simulink model "QDrone_YOLO_Recenter_Integration_Test"  (R2021b)
settings: Solver=ode2  StartTime=0.0  StopTime=60  FixedStep=0.001  RelTol=1e-3  EnableMultiTasking=on
undefined symbols (not defined in the file): Host, qc_get_step_size
libraries: quarc_library x32, simulink x5, dspnetwork x1
(part 1 of 2)
settings Model: SimulationMode=external  ExtModeTrigDuration=10000  Creator=Admin  LastModifiedBy=user
settings SolverCC: AlgebraicLoopSolver=TrustRegion  PositivePriorityOrder=on
settings DataIOCC: ReturnWorkspaceOutputs=off
settings DebuggingCC: SFUnexpectedBacktrackingDiag=warning  SFNoUnconditionalDefaultTransitionDiag=warning  SFExecutionAtInitializationDiag=none  SFMachineParentedDataDiag=warning  ArithmeticOperatorsInVariantConditions=warning
settings SFSimCC: SimUseLocalCustomCode=off  CustomCodeUndefinedFunction=UseInterfaceOnly
settings RTWCC: Description=QUARC Win64 Target Using Toolchain  SystemTargetFile=quarc_win64.tlc  TemplateMakefile=quarc_default_tmf  RTWUseLocalCustomCode=off  Toolchain=QUARC win64 | nmake (64-bit Windows)  BuildConfiguration=Faster Runs
settings CodeAppCC: StateflowObjectComments=on
settings STFCustomTargetCC: ConcurrentExecutionCompliant=on  UseToolchainInfoCompliant=on  SystemTargetFile=quarc_win64.tlc
settings GRTTargetCC: TargetLangStandard=C89/C90 (ANSI)  ParMdlRefBuildCompliant=off  CompOptLevelCompliant=off  CombineOutputUpdateFcns=off  MatFileLogging=off  CPPClassGenCompliant=off  GRTInterface=on  ExtMode=on  ExtModeMexFile=quarc_comm  ExtModeMexArgs='-w -d %d -uri %u -URI_Leader tcpip://localhost:18001 -URI_Follower tcpip://localhost:18002'
settings ConfigComp: CovMetricSettings=dw  CovSaveCumulativeToWorkspaceVar=on  CovSaveSingleToWorkspaceVar=on  CovExternalEMLEnable=off

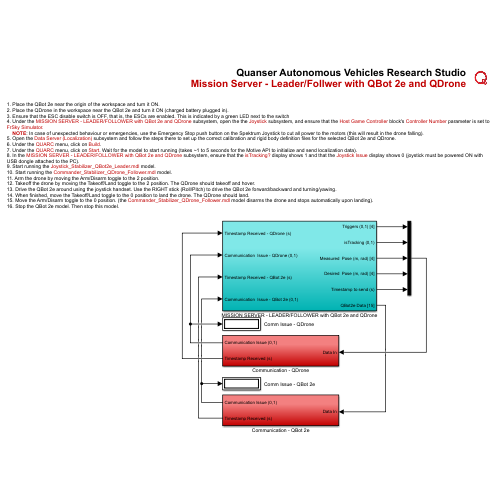
[thumbnail: Simulink's stored preview of the top-level diagram]
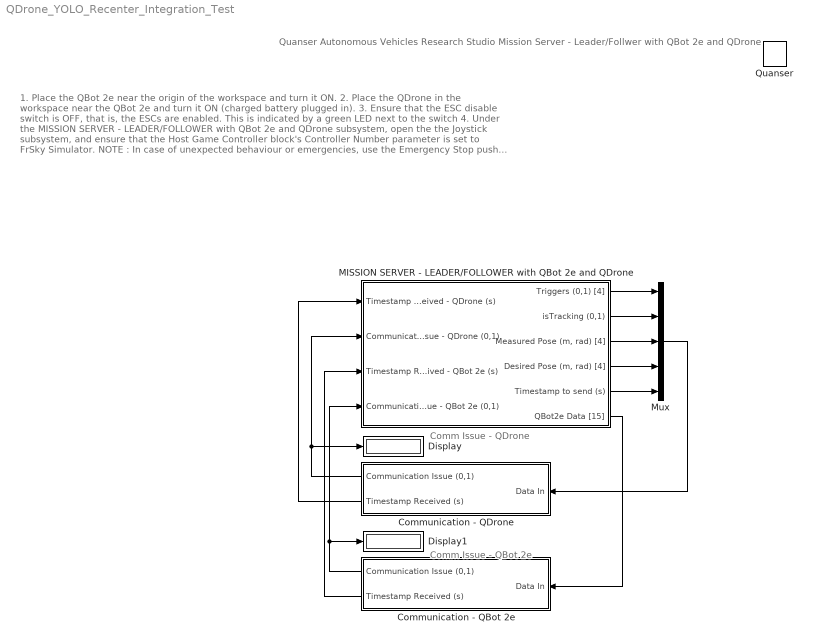
== system QDrone_YOLO_Recenter_Integration_Test ==
  note: 1. Place the QBot 2e near the origin of the workspace and turn it ON.
      | 2. Place the QDrone in the workspace near the QBot 2e and turn it ON (charged battery plugged in).
      | 3. Ensure that the ESC disable switch is OFF, that is, the ESCs are enabled. This is indicated by a green LED next to the switch
      | 4. Under the MISSION SERVER - LEADER/FOLLOWER with QBot 2e and QDrone subsystem, open the the Joystick subsystem, and ensure that the Host Game Controller block's Controller Number parameter is set to FrSky Simulator.
      | NOTE : In case of unexpected behaviour or emergencies, use the Emergency Stop push button on the Spektrum Joystick to cut all power to the motors (this will result in the drone falling).
      | 5. Open the Data Server (Localization) subsystem and follow the steps there to set up the correct calibration and rigid body definition files for the selected QBot 2e and QDrone.
      | 6. Under the QUARC menu, click on Build .
      | 7. Under the QUARC menu, click on Start . Wait for the model to start running (takes ~1 to 5 seconds for the Motive API to initialize and send localization data).
      | 8. In the MISSION SERVER - LEADER/FOLLOWER with QBot 2e and QDrone subsystem, ensure that the isTracking? display shows 1 and that the Joystick Issue display shows 0 (joystick must be powered ON with USB dongle attached to the PC).
      | 9. Start running the Joystick_Stabilizer_QBot2e_Leader.mdl model.
      | 10. Start running the Commander_Stabilizer_QDrone_Follower.mdl model.
      | 11. Arm the drone by moving the Arm/Disarm toggle to the 2 position.
      | 12. Takeoff the drone by moving the Takeoff/Land toggle to the 2 position. The QDrone should takeoff and hover.
      | 13. Drive the QBot 2e around using the joystick handset. Use the RIGHT stick (Roll/Pitch) to drive the QBot 2e forward/backward and turning/yawing.
      | 14. When finished, move the Takeoff/Land toggle to the 0 position to land the drone. The QDrone should land.
      | 15. Move the Arm/Disarm toggle to the 0 position. (the Commander_Stabilizer_QDrone_Follower.mdl model disarms the drone and stops automatically upon landing).
      | 16. Stop the QBot 2e model. Then stop this model.
  note: Quanser Autonomous Vehicles Research Studio
      | Mission Server - Leader/Follwer with QBot 2e and QDrone
  note: Comm Issue - QDrone
  note: Comm Issue - QBot 2e
  Communication - QBot 2e : Subsystem
  Communication - QDrone : Subsystem
  Display : Display
  Display1 : Display
  MISSION SERVER - LEADER/FOLLOWER with QBot 2e and QDrone : Subsystem
  Mux : Mux  Inputs=5
  Quanser : quarc_library/Logos/Quanser
  wires:
  Communication - QDrone/2(Timestamp Received (s)) -> MISSION SERVER - LEADER/FOLLOWER with QBot 2e and QDrone/1(Timestamp Received - QDrone (s))
  MISSION SERVER - LEADER/FOLLOWER with QBot 2e and QDrone/5(Timestamp to send (s)) -> Mux/5
  Mux/1 -> Communication - QDrone/1(Data In)
  Communication - QDrone/1(Communication Issue (0,1)) -> Display/1, MISSION SERVER - LEADER/FOLLOWER with QBot 2e and QDrone/2(Communication Issue - QDrone (0,1))
  MISSION SERVER - LEADER/FOLLOWER with QBot 2e and QDrone/3("Measured Pose (m, rad) [4]") -> Mux/3
  MISSION SERVER - LEADER/FOLLOWER with QBot 2e and QDrone/4("Desired Pose (m, rad) [4]") -> Mux/4
  Communication - QBot 2e/1(Communication Issue (0,1)) -> MISSION SERVER - LEADER/FOLLOWER with QBot 2e and QDrone/4(Communication Issue - QBot 2e (0,1)), Display1/1
  Communication - QBot 2e/2(Timestamp Received (s)) -> MISSION SERVER - LEADER/FOLLOWER with QBot 2e and QDrone/3(Timestamp Received - QBot 2e (s))
  MISSION SERVER - LEADER/FOLLOWER with QBot 2e and QDrone/6(QBot2e Data [15]) -> Communication - QBot 2e/1(Data In)
  MISSION SERVER - LEADER/FOLLOWER with QBot 2e and QDrone/1(Triggers (0,1) [4]) -> Mux/1
  MISSION SERVER - LEADER/FOLLOWER with QBot 2e and QDrone/2(isTracking (0,1)) -> Mux/2

== system QDrone_YOLO_Recenter_Integration_Test/Communication - QBot 2e ==
  note: Argument (URI_Leader) is set at the MEX-file arguments found at Model Configuration Properties > Code Generation > Interface
      |
      | Format:
      | tcpip://localhost:18001
  Data In : Inport
  Constant : Constant
  Detect Communication loss : Subsystem
  Model Argument : quarc_library/Sources/Signals/Model Argument  argument_name=URI_Leader  has_value=on  data_type_mode=Specify via dialog  data_type=char  max_length=80  default_value=0  variable_size=off
      settings: AttributesFormatString=(-%<argument_name>)  SourceProductName=QUARC Targets
  Stream Server : quarc_library/Communications/Basic/Stream Server  uri_source=External input port  uri=tcpip://localhost:18877  send_buffer_size=1460  receive_buffer_size=1460  byte_order=little endian (Intel - LSB first)  optimization=Minimum latency  send_options=Send most recent data  receive_options=Receive most recent data  default_value=[0]  sample_time=qc_get_step_size  active=off  implementation=Use blocking I/O in a separate thread  send_fifo_size=1000  receive_fifo_size=1000  send_priority=0  receive_priority=0  send_dimensions=off  receive_dimensions=off  max_dimensions=-1  data_type=Inherited via back propagation  type_expr=BusObject
  "String Display " : quarc_library/Strings/String Display  alignment=center  display_mode=Single line  sample_time=-1  use_new=off
      settings: SourceProductName=QUARC Targets
  Terminator1 : Terminator
  Terminator2 : Terminator
  Communication Issue (0,1) : Outport  VectorParamsAs1DForOutWhenUnconnected=off
  Timestamp Received (s) : Outport  Port=2  VectorParamsAs1DForOutWhenUnconnected=off
  wires:
  Detect Communication loss/1(Communication Issue (0,1)) -> Communication Issue (0,1)/1
  Stream Server/2 -> Detect Communication loss/2(Error)
  Stream Server/1 -> Detect Communication loss/1(State)
  Stream Server/4 -> Timestamp Received (s)/1
  Model Argument/1 -> Stream Server/3, "String Display "/1
  Stream Server/5 -> Terminator1/1
  Stream Server/3 -> Terminator2/1
  Constant/1 -> Stream Server/2
  Data In/1 -> Stream Server/1

== system QDrone_YOLO_Recenter_Integration_Test/Communication - QDrone ==
  note: Argument (URI_Follower) is set at the MEX-file arguments found at Model Configuration Properties > Code Generation > Interface
      |
      | Format:
      | tcpip://localhost:18002
  Data In : Inport
  Constant : Constant
  Detect Communication loss : Subsystem
  Model Argument : quarc_library/Sources/Signals/Model Argument  argument_name=URI_Follower  has_value=on  data_type_mode=Specify via dialog  data_type=char  max_length=80  default_value=0  variable_size=off
      settings: AttributesFormatString=(-%<argument_name>)  SourceProductName=QUARC Targets
  Stream Server : quarc_library/Communications/Basic/Stream Server  uri_source=External input port  uri=tcpip://localhost:18877  send_buffer_size=1460  receive_buffer_size=1460  byte_order=little endian (Intel - LSB first)  optimization=Minimum latency  send_options=Send most recent data  receive_options=Receive most recent data  default_value=zeros(1,1)  sample_time=qc_get_step_size  active=off  implementation=Use blocking I/O in a separate thread  send_fifo_size=1000  receive_fifo_size=1000  send_priority=0  receive_priority=0  send_dimensions=off  receive_dimensions=off  max_dimensions=-1  data_type=Inherited via back propagation  type_expr=BusObject
  "String Display " : quarc_library/Strings/String Display  alignment=center  display_mode=Single line  sample_time=-1  use_new=off
      settings: SourceProductName=QUARC Targets
  Terminator1 : Terminator
  Terminator2 : Terminator
  Communication Issue (0,1) : Outport  VectorParamsAs1DForOutWhenUnconnected=off
  Timestamp Received (s) : Outport  Port=2  VectorParamsAs1DForOutWhenUnconnected=off
  wires:
  Constant/1 -> Stream Server/2
  Data In/1 -> Stream Server/1
  Stream Server/3 -> Terminator2/1
  Stream Server/5 -> Terminator1/1
  Model Argument/1 -> "String Display "/1, Stream Server/3
  Stream Server/4 -> Timestamp Received (s)/1
  Stream Server/1 -> Detect Communication loss/1(State)
  Stream Server/2 -> Detect Communication loss/2(Error)
  Detect Communication loss/1(Communication Issue (0,1)) -> Communication Issue (0,1)/1

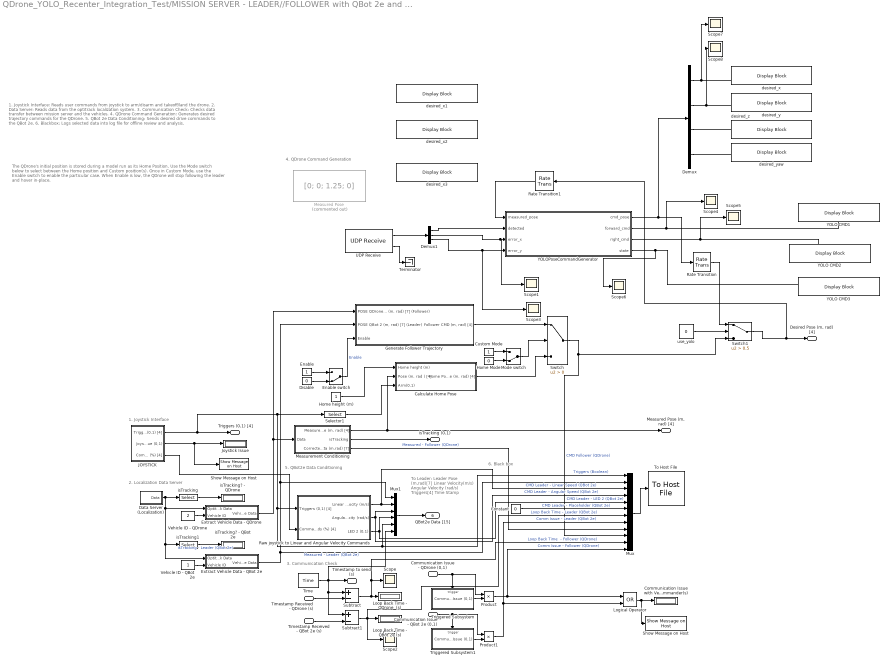
== system QDrone_YOLO_Recenter_Integration_Test/MISSION SERVER - LEADER//FOLLOWER with QBot 2e and QDrone ==
  note: To Leader:
      | Leader Pose (m,rad)[7]
      | Linear Velocity(m/s)
      | Angular Velocity (rad/s)
      | Triggers[4]
      | Time Stamp
  note: 5. QBot2e Data Conditioning
  note: The QDrone's initial position is stored during a model run as its Home Position.
      | Use the Mode switch below to select between the Home position and Custom position(s).
      | Once in Custom Mode, use the Enable switch to enable the particular case.
      | When Enable is low, the QDrone will stop following the leader and hover in-place.
  note: 3. Communication Check
  note: 6. Black box
  note: 2. Localization Data Server
  note: 1. Joystick Interface
  note: 4. QDrone Command Generation
  note: 1. Joystick Interface: Reads user commands from joystick to arm/disarm and takeoff/land the drone.
      | 2. Data Server: Reads data from the optitrack localization system.
      | 3. Communication Check: Checks data transfer between mission server and the vehicles.
      | 4. QDrone Command Generation: Generates desired trajectory commands for the QDrone.
      | 5. QBot 2e Data Conditioning: Sends desired drive commands to the QBot 2e.
      | 6. Blackbox: Logs selected data into log file for offline review and analysis.
  Timestamp Received - QDrone (s) : Inport
  Communication Issue - QDrone (0,1) : Inport  Port=2
  Timestamp Received - QBot 2e (s) : Inport  Port=3
  Communication Issue - QBot 2e (0,1) : Inport  Port=4
   desired_x{,1..3} (4 alike) : DisplayBlock  LabelPosition=Hide  Format=short  Transparency=1
  Calculate Home Pose : Subsystem
  Communication Issue with Vehicle Commander(s) : Display
  Constant : Constant  Value=0
  Custom Mode : Constant
  "Data Server (Localization) " : Subsystem
  Demux : Demux
  Demux1 : Demux  Outputs=3
  Disable : Constant  Value=0
  Enable : Constant
  Enable switch : ManualSwitch  CurrentSetting=0
  Extract Vehicle Data - QBot 2e : Subsystem
  Extract Vehicle Data - QDrone : Subsystem
  Generate Follower Trajectory : Subsystem
  Home Mode : Constant  Value=0
  Home height (m) : Constant
  JOYSTICK : Subsystem
  Joystick Issue : Display
  Logical Operator : Logic  Operator=OR  AllPortsSameDT=off  OutDataTypeStr=boolean
  Loop Back Time - QBot 2e (s) : Display
  Loop Back Time - QDrone  (s) : Display
  Measured Pose : Constant  Commented=on  Value=[0; 0; 1.25; 0]  OutDataTypeStr=double
  Measurement Conditioning : Subsystem
  Mode switch : ManualSwitch  CurrentSetting=0
  Mux : Mux  Inputs=12
  Mux1 : Mux  Inputs=6
  Product : Product
  Product1 : Product
  Rate Transition : RateTransition  OutPortSampleTime=0.001
  Rate Transition1 : RateTransition  OutPortSampleTime=0.033
  Raw joystick to Linear and Angular Velocity Commands : Subsystem
  Scope{,1..8} (9 alike) : Scope
  Selector1 : Selector  InputPortWidth=4  IndexOptions=Index vector (dialog)  Indices=[1]  OutputSizes=1
  Show Message on Host : quarc_library/Sinks/Error Handling/Show Message on Host  message_type=Fixed error message  message_icon=Warning  message=Mission Server: Communication Issue with remote vehicle(s)
      settings: AttributesFormatString="\"%<message>\""  SourceProductName=QUARC Targets
  "Show Message on Host " : quarc_library/Sinks/Error Handling/Show Message on Host  message_type=Fixed error message  message_icon=Warning  message=Mission Server: Joystick Disconnected
      settings: AttributesFormatString="\"%<message>\""  SourceProductName=QUARC Targets
  Subtract : Sum  Inputs=+-
  Subtract1 : Sum  Inputs=+-
  Switch : Switch  Criteria=u2 > Threshold
  Switch1 : Switch  Criteria=u2 > Threshold  Threshold=0.5
  Terminator : Terminator
  Time : quarc_library/Sources/Time/Time  time_source=Wall clock  sample_time=qc_get_step_size
  To Host File : quarc_library/Sinks/To Host/To Host File  file_name=saved_data/%m/Mission_Server_%{date}_%{time}.mat  variable_name=mission_server_data  decimation=1  sample_time=-1  file_format=MAT-file v.5  options=No header or footer  append=off  final_file_name=saved_data/QDrone_YOLO_Recenter_Integration_Test/Mission_Server_03-Jun-2026_14-38-11.mat  bitrate=2000000
  Triggered Subsystem : Subsystem  TreatAsAtomicUnit=on
  Triggered Subsystem1 : Subsystem  TreatAsAtomicUnit=on
  UDP Receive : dspnetwork/UDP Receive  localURL='0.0.0.0'  localPort=5010  remoteURL='0.0.0.0'  remotePort=-1  recvBufferSize=8192  dims=3  signalDatatype=double  isComplex=off  isVarSize=off  showBlockingTime=off  blockingTime=0  sampletime=0.033  blockPlatform=[]
  Vehicle ID - QBot 2e : Constant
  Vehicle ID - QDrone : Constant  Value=2
  YOLO CMD1 : DisplayBlock  LabelPosition=Hide  Format=short  Transparency=1
  YOLO CMD2 : DisplayBlock  LabelPosition=Hide  Format=short  Transparency=1
  YOLO CMD3 : DisplayBlock  LabelPosition=Hide  Format=short  Transparency=1
  YOLOPoseCommandGenerator : MATLAB Function  TreatAsAtomicUnit=on
  desired_y : DisplayBlock  LabelPosition=Hide  Format=short  Transparency=1
  "desired_yaw " : DisplayBlock  LabelPosition=Hide  Format=short  Transparency=1
  "desired_z " : DisplayBlock  LabelPosition=Hide  Format=short  Transparency=1
  isTracking : Selector  InputPortWidth=14  IndexOptions=Index vector (dialog)  Indices=[14]  OutputSizes=1
  isTracking1 : Selector  InputPortWidth=14  IndexOptions=Index vector (dialog)  Indices=[13]  OutputSizes=1
  isTracking? - QBot 2e : Display
  isTracking? - QDrone : Display
  use_yolo : Constant  Value=0
  Triggers (0,1) [4] : Outport  VectorParamsAs1DForOutWhenUnconnected=off
  isTracking (0,1) : Outport  Port=2  VectorParamsAs1DForOutWhenUnconnected=off
  "Measured Pose (m, rad) [4]" : Outport  Port=3  VectorParamsAs1DForOutWhenUnconnected=off
  "Desired Pose (m, rad) [4]" : Outport  Port=4  VectorParamsAs1DForOutWhenUnconnected=off
  Timestamp to send (s) : Outport  Port=5  VectorParamsAs1DForOutWhenUnconnected=off
  QBot2e Data [15] : Outport  Port=6  VectorParamsAs1DForOutWhenUnconnected=off
  wires:
  Communication Issue - QDrone (0,1)/1 -> Product/1, Triggered Subsystem/Trigger
  isTracking/1 -> isTracking? - QDrone/1
  JOYSTICK/2(Joystick Issue (0,1)) -> Joystick Issue/1, "Show Message on Host "/1
  Time/1 -> Mux1/6, Subtract1/1, Subtract/1, Timestamp to send (s)/1
  Timestamp Received - QDrone (s)/1 -> Subtract/2
  Subtract/1 -> Mux/11, Scope/1, Loop Back Time - QDrone  (s)/1  "Loop Back Time  - Follower (QDrone)"
  Switch/1 -> Mux/10, Switch1/3  "CMD Follower (QDrone)"
  Measurement Conditioning/2(isTracking) -> isTracking (0,1)/1
  Measurement Conditioning/1("Measured Pose (m, rad) [4]") -> "Measured Pose (m, rad) [4]"/1, Calculate Home Pose/2("Pose (m, rad ) [4]")
  "Data Server (Localization) "/1(Data) -> isTracking1/1, Extract Vehicle Data - QBot 2e/1(Optitrack Data), Extract Vehicle Data - QDrone/1(Optitrack Data), isTracking/1
  Vehicle ID - QDrone/1 -> Extract Vehicle Data - QDrone/2(Vehicle ID)
  Calculate Home Pose/1("Home Pose (m, rad) [4]") -> Switch/3
  Home height (m)/1 -> Calculate Home Pose/1(Home height (m))
  Triggered Subsystem/1(Communication Issue (0,1)) -> Product/2
  Product/1 -> Logical Operator/1, Mux/12  "Comm Issue - Follower (QDrone)"
  Mux/1 -> To Host File/1
  Custom Mode/1 -> Mode switch/1
  Mode switch/1 -> Switch/2
  Home Mode/1 -> Mode switch/2
  Enable/1 -> Enable switch/1
  Disable/1 -> Enable switch/2
  Enable switch/1 -> Generate Follower Trajectory/3(Enable)  "Enable"
  Generate Follower Trajectory/1("Follower CMD (m, rad) [4]") -> Switch/1
  Vehicle ID - QBot 2e/1 -> Extract Vehicle Data - QBot 2e/2(Vehicle ID)
  Timestamp Received - QBot 2e (s)/1 -> Subtract1/2
  Subtract1/1 -> Mux/7, Loop Back Time - QBot 2e (s)/1, Scope2/1  "Loop Back Time - Leader (QBot 2e)"
  Logical Operator/1 -> Show Message on Host/1, Communication Issue with Vehicle Commander(s)/1
  Product1/1 -> Logical Operator/2, Mux/8  "Comm Issue - Leader (QBot 2e)"
  Triggered Subsystem1/1(Communication Issue (0,1)) -> Product1/2
  Communication Issue - QBot 2e (0,1)/1 -> Product1/1, Triggered Subsystem1/Trigger
  Extract Vehicle Data - QBot 2e/1(Vehicle Data) -> Mux/2, Generate Follower Trajectory/2("POSE QBot 2 (m, rad) [7] (Leader)"), Mux1/1  "Measured - Leader (QBot 2e)"
  Extract Vehicle Data - QDrone/1(Vehicle Data) -> Measurement Conditioning/1(Data), Generate Follower Trajectory/1("POSE QDrone (m, rad) [7] (Follower)")
  isTracking1/1 -> isTracking? - QBot 2e/1  "isTracking - Leader (QBot 2e)"
  JOYSTICK/1(Triggers (0,1) [4]) -> Triggers (0,1) [4]/1, Selector1/1, Raw joystick to Linear and Angular Velocity Commands/1(Triggers (0,1) [4]), Mux/1, Mux1/5  "Triggers (Boolean)"
  Mux1/1 -> QBot2e Data [15]/1
  JOYSTICK/3(Commands (%) [4]) -> Raw joystick to Linear and Angular Velocity Commands/2(Commands (%) [4])
  Raw joystick to Linear and Angular Velocity Commands/1(Linear Velocity (m/s)) -> Mux/3, Mux1/2  "CMD Leader - Linear Speed (QBot 2e)"
  Raw joystick to Linear and Angular Velocity Commands/2(Angular Velocity (rad/s)) -> Mux1/3, Mux/4  "CMD Leader - Angular Speed (QBot 2e)"
  Raw joystick to Linear and Angular Velocity Commands/3(LED 2 (0,1)) -> Mux/5, Mux1/4  "CMD Leader - LED 2 (QBot 2e)"
  Selector1/1 -> Calculate Home Pose/3(Arm(0,1))
  Measurement Conditioning/3(Corrected Pose Data (m,rad) [7]) -> Mux/9  "Measured - Follower (QDrone)"
  Constant/1 -> Mux/6  "CMD Leader - Placeholder (QBot 2e)"
  Demux/4 -> ?
  Demux/2 -> Scope8/1
  Demux/3 -> ?
  YOLOPoseCommandGenerator/1(cmd_pose) -> Demux/1, Rate Transition/1
  use_yolo/1 -> Switch1/2
  Switch1/1 -> Rate Transition1/1, "Desired Pose (m, rad) [4]"/1
  UDP Receive/1 -> Demux1/1
  Demux1/2 -> YOLOPoseCommandGenerator/3(error_x), Scope1/1
  Demux1/3 -> YOLOPoseCommandGenerator/4(error_y), Scope3/1
  UDP Receive/2 -> Terminator/1
  Rate Transition/1 -> Switch1/1
  Rate Transition1/1 -> YOLOPoseCommandGenerator/1(measured_pose)
  YOLOPoseCommandGenerator/2(forward_cmd) -> Scope4/1
  YOLOPoseCommandGenerator/3(right_cmd) -> Scope5/1
  YOLOPoseCommandGenerator/4(state) -> Scope6/1
  Demux/1 -> Scope7/1
  Demux1/1 -> YOLOPoseCommandGenerator/2(detected)

== system QDrone_YOLO_Recenter_Integration_Test/Communication - QBot 2e/Detect Communication loss ==
  note: Check if stream is 2 (connected) and error is positive (error codes are negative). Otherwise issue a communication error.
  State : Inport
  Error : Inport  Port=2
  Data Type Conversion : DataTypeConversion
  MATLAB Function : MATLAB Function  TreatAsAtomicUnit=on
  Terminator2 : Terminator
  Threshold : quarc_library/Discontinuities/Threshold  operator=>=  param_src=Specify via dialog  threshold=0.5  duration=0.1
      settings: SourceProductName=QUARC Targets
  Time : quarc_library/Sources/Time/Time  time_source=Wall clock  sample_time=qc_get_step_size
  Communication Issue (0,1) : Outport  VectorParamsAs1DForOutWhenUnconnected=off
  wires:
  Threshold/1 -> Data Type Conversion/1
  Data Type Conversion/1 -> Communication Issue (0,1)/1
  Threshold/2 -> Terminator2/1
  Time/1 -> MATLAB Function/1(time)
  State/1 -> MATLAB Function/2(state)
  MATLAB Function/1(stream_connection_loss) -> Threshold/1
  Error/1 -> MATLAB Function/3(error)

== system QDrone_YOLO_Recenter_Integration_Test/Communication - QDrone/Detect Communication loss ==
  note: Check if stream is 2 (connected) and error is positive (error codes are negative). Otherwise issue a communication error.
  State : Inport
  Error : Inport  Port=2
  Data Type Conversion : DataTypeConversion
  MATLAB Function : MATLAB Function  TreatAsAtomicUnit=on
  Terminator2 : Terminator
  Threshold : quarc_library/Discontinuities/Threshold  operator=>=  param_src=Specify via dialog  threshold=0.5  duration=0.1
      settings: SourceProductName=QUARC Targets
  Time : quarc_library/Sources/Time/Time  time_source=Wall clock  sample_time=qc_get_step_size
  Communication Issue (0,1) : Outport  VectorParamsAs1DForOutWhenUnconnected=off
  wires:
  Error/1 -> MATLAB Function/3(error)
  MATLAB Function/1(stream_connection_loss) -> Threshold/1
  State/1 -> MATLAB Function/2(state)
  Time/1 -> MATLAB Function/1(time)
  Threshold/2 -> Terminator2/1
  Data Type Conversion/1 -> Communication Issue (0,1)/1
  Threshold/1 -> Data Type Conversion/1

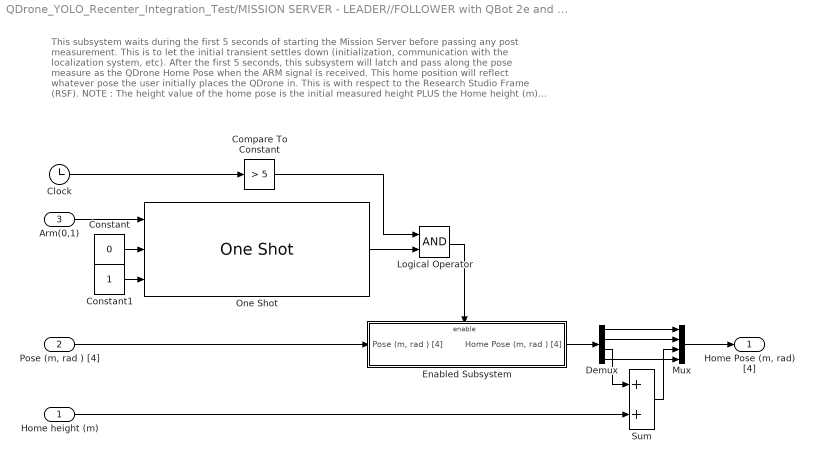
== system QDrone_YOLO_Recenter_Integration_Test/MISSION SERVER - LEADER//FOLLOWER with QBot 2e and QDrone/Calculate Home Pose ==
  note: This subsystem waits during the first 5 seconds of starting the Mission Server before passing any post measurement.
      | This is to let the initial transient settles down (initialization, communication with the localization system, etc).
      | After the first 5 seconds, this subsystem will latch and pass along the pose measure as the QDrone Home Pose when
      | the ARM signal is received.
      | This home position will reflect whatever pose the user initially places the QDrone in.
      | This is with respect to the Research Studio Frame (RSF).
      |
      | NOTE : The height value of the home pose is the initial measured height PLUS the Home height (m) input value.
  Home height (m) : Inport
  "Pose (m, rad ) [4]" : Inport  Port=2
  Arm(0,1) : Inport  Port=3
  Clock : Clock
  Compare To Constant : simulink/Logic and Bit Operations/Compare To Constant  relop=>  const=5  OutDataTypeStr=boolean
  Constant : Constant  Value=0
  Constant1 : Constant
  Demux : Demux
  Enabled Subsystem : Subsystem  TreatAsAtomicUnit=on
  Logical Operator : Logic  AllPortsSameDT=off  OutDataTypeStr=boolean
  Mux : Mux
  One Shot : quarc_library/Discontinuities/One Shot  trigger_type=Rising edge  redun_pulse=Ignore extraneous pulse  width_source=Specify via dialog  pulse_width=1/qc_get_step_size
      settings: SourceProductName=QUARC Targets
  Sum : Sum
  "Home Pose (m, rad) [4]" : Outport  VectorParamsAs1DForOutWhenUnconnected=off
  wires:
  Constant/1 -> One Shot/2
  Constant1/1 -> One Shot/3
  Arm(0,1)/1 -> One Shot/1
  One Shot/1 -> Logical Operator/2
  "Pose (m, rad ) [4]"/1 -> Enabled Subsystem/1("Pose (m, rad ) [4] ")
  Clock/1 -> Compare To Constant/1
  Compare To Constant/1 -> Logical Operator/1
  Logical Operator/1 -> Enabled Subsystem/Enable
  Enabled Subsystem/1("Home Pose (m, rad ) [4]") -> Demux/1
  Demux/1 -> Mux/1
  Demux/2 -> Mux/2
  Demux/4 -> Mux/4
  Demux/3 -> Sum/1
  Sum/1 -> Mux/3
  Home height (m)/1 -> Sum/2
  Mux/1 -> "Home Pose (m, rad) [4]"/1

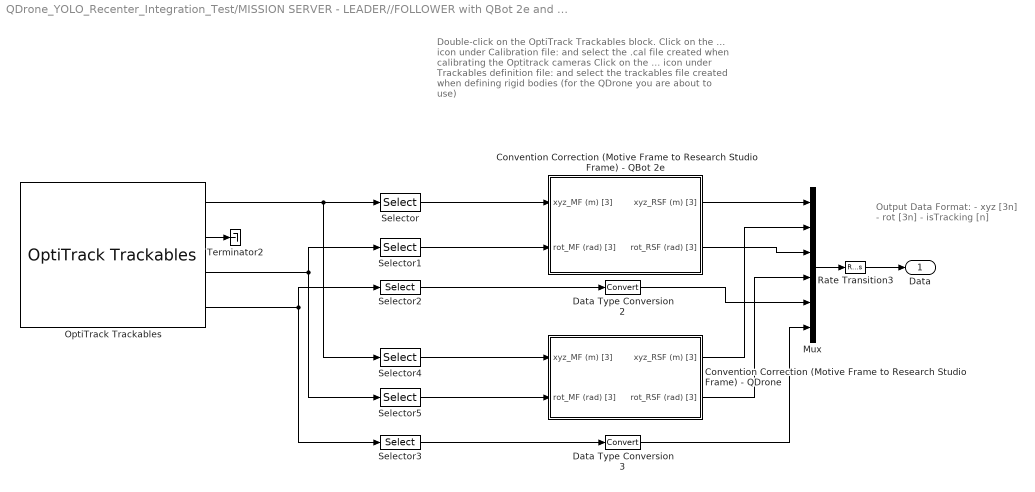
== system QDrone_YOLO_Recenter_Integration_Test/MISSION SERVER - LEADER//FOLLOWER with QBot 2e and QDrone/Data Server (Localization)  ==
  note: Output Data Format:
      | - xyz [3n]
      | - rot [3n]
      | - isTracking [n]
  note: Double-click on the OptiTrack Trackables block.
      |
      | Click on the ... icon under Calibration file: and select the .cal file
      | created when calibrating the Optitrack cameras
      |
      | Click on the ... icon under Trackables definition file: and select
      | the trackables file created when defining rigid bodies (for the
      | QDrone you are about to use)
  Convention Correction (Motive Frame to Research Studio Frame) - QBot 2e : Subsystem
  Convention Correction (Motive Frame to Research Studio Frame) - QDrone : Subsystem
  Data Type Conversion2 : DataTypeConversion
  Data Type Conversion3 : DataTypeConversion
  Mux : Mux  Inputs=6
  OptiTrack Trackables : quarc_library/Devices/Third-Party/NaturalPoint/OptiTrack/OptiTrack Trackables  calibration_file=C:\Users\user\Documents\OptiTrack\2023-05-04\Calibration Exceptional (MeanErr 0.642 mm) 2023-05-04 12.cal  rigid_body_file=C:\Users\user\Documents\OptiTrack\2023-05-04\RigidBody 02.tra  rigid_body_ids=[1,2]  sample_time=qc_get_step_size*10  active=off
      settings: SourceProductName=QUARC Targets
  Rate Transition3 : RateTransition
  Selector : Selector  InputPortWidth=6  IndexOptions=Index vector (dialog)  Indices=[1:3]  OutputSizes=1
  Selector1 : Selector  InputPortWidth=6  IndexOptions=Index vector (dialog)  Indices=[1:3]  OutputSizes=1
  Selector2 : Selector  InputPortWidth=2  IndexOptions=Index vector (dialog)  Indices=[1]  OutputSizes=1
  Selector3 : Selector  InputPortWidth=2  IndexOptions=Index vector (dialog)  Indices=[2]  OutputSizes=1
  Selector4 : Selector  InputPortWidth=6  IndexOptions=Index vector (dialog)  Indices=[4:6]  OutputSizes=1
  Selector5 : Selector  InputPortWidth=6  IndexOptions=Index vector (dialog)  Indices=[4:6]  OutputSizes=1
  Terminator2 : Terminator
  Data : Outport  VectorParamsAs1DForOutWhenUnconnected=off
  wires:
  Convention Correction (Motive Frame to Research Studio Frame) - QBot 2e/1(xyz_RSF (m) [3]) -> Mux/1
  Data Type Conversion2/1 -> Mux/5
  Convention Correction (Motive Frame to Research Studio Frame) - QBot 2e/2(rot_RSF (rad) [3]) -> Mux/3
  OptiTrack Trackables/2 -> Terminator2/1
  Data Type Conversion3/1 -> Mux/6
  Convention Correction (Motive Frame to Research Studio Frame) - QDrone/2(rot_RSF (rad) [3]) -> Mux/4
  OptiTrack Trackables/4 -> Selector2/1, Selector3/1
  Convention Correction (Motive Frame to Research Studio Frame) - QDrone/1(xyz_RSF (m) [3]) -> Mux/2
  OptiTrack Trackables/3 -> Selector5/1, Selector1/1
  Selector1/1 -> Convention Correction (Motive Frame to Research Studio Frame) - QBot 2e/2(rot_MF (rad) [3])
  Selector2/1 -> Data Type Conversion2/1
  Selector3/1 -> Data Type Conversion3/1
  OptiTrack Trackables/1 -> Selector4/1, Selector/1
  Selector/1 -> Convention Correction (Motive Frame to Research Studio Frame) - QBot 2e/1(xyz_MF (m) [3])
  Selector4/1 -> Convention Correction (Motive Frame to Research Studio Frame) - QDrone/1(xyz_MF (m) [3])
  Selector5/1 -> Convention Correction (Motive Frame to Research Studio Frame) - QDrone/2(rot_MF (rad) [3])
  Mux/1 -> Rate Transition3/1
  Rate Transition3/1 -> Data/1

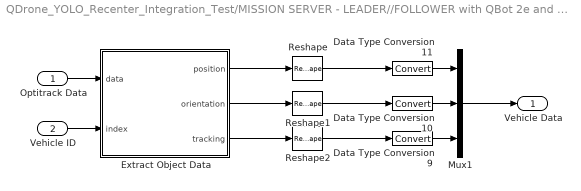
== system QDrone_YOLO_Recenter_Integration_Test/MISSION SERVER - LEADER//FOLLOWER with QBot 2e and QDrone/Extract Vehicle Data - QBot 2e ==
  Optitrack Data : Inport
  Vehicle ID : Inport  Port=2
  Data Type Conversion10 : DataTypeConversion
  Data Type Conversion11 : DataTypeConversion
  Data Type Conversion9 : DataTypeConversion
  Extract Object Data : MATLAB Function  TreatAsAtomicUnit=on
  Mux1 : Mux  Inputs=3
  Reshape : Reshape
  Reshape1 : Reshape
  Reshape2 : Reshape
  Vehicle Data : Outport  VectorParamsAs1DForOutWhenUnconnected=off
  wires:
  Reshape2/1 -> Data Type Conversion9/1
  Reshape1/1 -> Data Type Conversion10/1
  Reshape/1 -> Data Type Conversion11/1
  Data Type Conversion9/1 -> Mux1/3
  Data Type Conversion10/1 -> Mux1/2
  Data Type Conversion11/1 -> Mux1/1
  Extract Object Data/2(orientation) -> Reshape1/1
  Extract Object Data/3(tracking) -> Reshape2/1
  Extract Object Data/1(position) -> Reshape/1
  Mux1/1 -> Vehicle Data/1
  Optitrack Data/1 -> Extract Object Data/1(data)
  Vehicle ID/1 -> Extract Object Data/2(index)

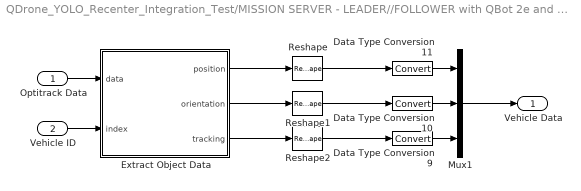
== system QDrone_YOLO_Recenter_Integration_Test/MISSION SERVER - LEADER//FOLLOWER with QBot 2e and QDrone/Extract Vehicle Data - QDrone ==
  Optitrack Data : Inport
  Vehicle ID : Inport  Port=2
  Data Type Conversion10 : DataTypeConversion
  Data Type Conversion11 : DataTypeConversion
  Data Type Conversion9 : DataTypeConversion
  Extract Object Data : MATLAB Function  TreatAsAtomicUnit=on
  Mux1 : Mux  Inputs=3
  Reshape : Reshape
  Reshape1 : Reshape
  Reshape2 : Reshape
  Vehicle Data : Outport  VectorParamsAs1DForOutWhenUnconnected=off
  wires:
  Reshape2/1 -> Data Type Conversion9/1
  Reshape1/1 -> Data Type Conversion10/1
  Reshape/1 -> Data Type Conversion11/1
  Data Type Conversion9/1 -> Mux1/3
  Data Type Conversion10/1 -> Mux1/2
  Data Type Conversion11/1 -> Mux1/1
  Extract Object Data/2(orientation) -> Reshape1/1
  Extract Object Data/3(tracking) -> Reshape2/1
  Extract Object Data/1(position) -> Reshape/1
  Mux1/1 -> Vehicle Data/1
  Optitrack Data/1 -> Extract Object Data/1(data)
  Vehicle ID/1 -> Extract Object Data/2(index)

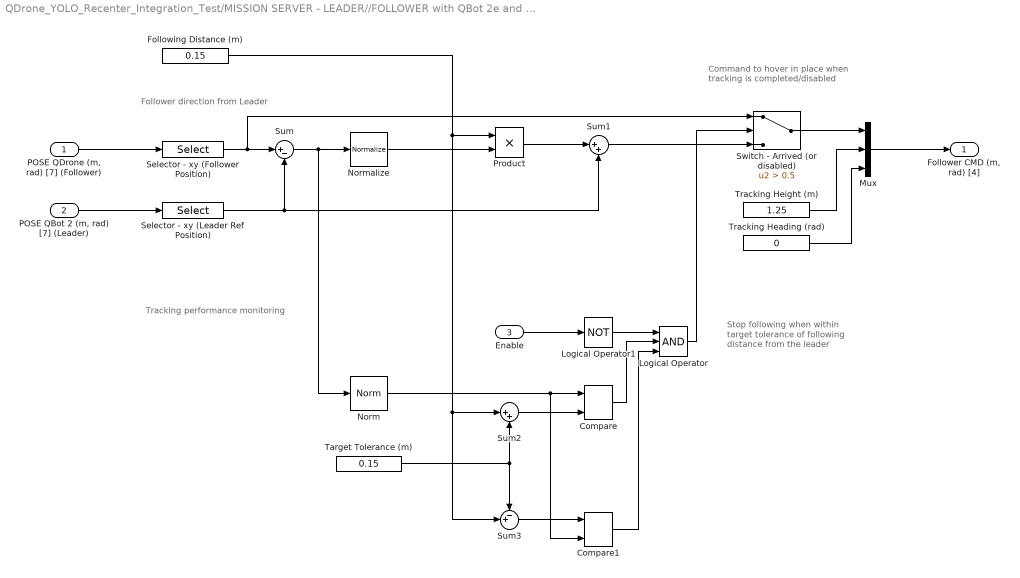
== system QDrone_YOLO_Recenter_Integration_Test/MISSION SERVER - LEADER//FOLLOWER with QBot 2e and QDrone/Generate Follower Trajectory ==
  note: Command to hover in place when
      | tracking is completed/disabled
  note: Stop following when
      | within target tolerance
      | of following distance from
      | the leader
  note: Tracking performance monitoring
  note: Follower direction from Leader
  "POSE QDrone (m, rad) [7] (Follower)" : Inport
  "POSE QBot 2 (m, rad) [7] (Leader)" : Inport  Port=2
  Enable : Inport  Port=3
  Compare : quarc_library/Logic Operations/Compare  operator=<=  output_data_type=boolean
      settings: SourceProductName=QUARC Targets
  Compare1 : quarc_library/Logic Operations/Compare  operator=>=  output_data_type=boolean
      settings: SourceProductName=QUARC Targets
  Following Distance (m) : Constant  Value=0.15
  Logical Operator : Logic  Inputs=3  AllPortsSameDT=off  OutDataTypeStr=boolean
  Logical Operator1 : Logic  Operator=NOT  Inputs=1  AllPortsSameDT=off  OutDataTypeStr=boolean
  Mux : Mux  Inputs=3
  Norm : quarc_library/Math Operations/Vectors/Norm
      settings: SourceProductName=QUARC Targets
  Normalize : quarc_library/Math Operations/Vectors/Normalize
      settings: SourceProductName=QUARC Targets
  Product : Product
  Selector - xy (Follower Position) : Selector  InputPortWidth=7  IndexOptions=Index vector (dialog)  Indices=[1 2]  OutputSizes=1
  Selector - xy (Leader Ref Position) : Selector  InputPortWidth=7  IndexOptions=Index vector (dialog)  Indices=[1 2]  OutputSizes=1
  Sum : Sum  Inputs=|+-
  Sum1 : Sum  Inputs=|++
  Sum2 : Sum  Inputs=|++
  Sum3 : Sum  Inputs=-+|
  Switch - Arrived (or disabled) : Switch  Criteria=u2 > Threshold  Threshold=0.5
  Target Tolerance (m) : Constant  Value=0.15
  Tracking Heading (rad) : Constant  Value=0
  Tracking Height (m) : Constant  Value=1.25
  "Follower CMD (m, rad) [4]" : Outport  VectorParamsAs1DForOutWhenUnconnected=off
  wires:
  "POSE QDrone (m, rad) [7] (Follower)"/1 -> Selector - xy (Follower Position)/1
  "POSE QBot 2 (m, rad) [7] (Leader)"/1 -> Selector - xy (Leader Ref Position)/1
  Selector - xy (Follower Position)/1 -> Switch - Arrived (or disabled)/1, Sum/1
  Selector - xy (Leader Ref Position)/1 -> Sum1/2, Sum/2
  Sum/1 -> Norm/1, Normalize/1
  Product/1 -> Sum1/1
  Normalize/1 -> Product/2
  Following Distance (m)/1 -> Product/1, Sum2/1, Sum3/2
  Tracking Height (m)/1 -> Mux/2
  Tracking Heading (rad)/1 -> Mux/3
  Sum1/1 -> Switch - Arrived (or disabled)/3
  Switch - Arrived (or disabled)/1 -> Mux/1
  Mux/1 -> "Follower CMD (m, rad) [4]"/1
  Sum2/1 -> Compare/2
  Sum3/1 -> Compare1/1
  Target Tolerance (m)/1 -> Sum2/2, Sum3/1
  Norm/1 -> Compare1/2, Compare/1
  Enable/1 -> Logical Operator1/1
  Logical Operator1/1 -> Logical Operator/1
  Compare/1 -> Logical Operator/2
  Compare1/1 -> Logical Operator/3
  Logical Operator/1 -> Switch - Arrived (or disabled)/2

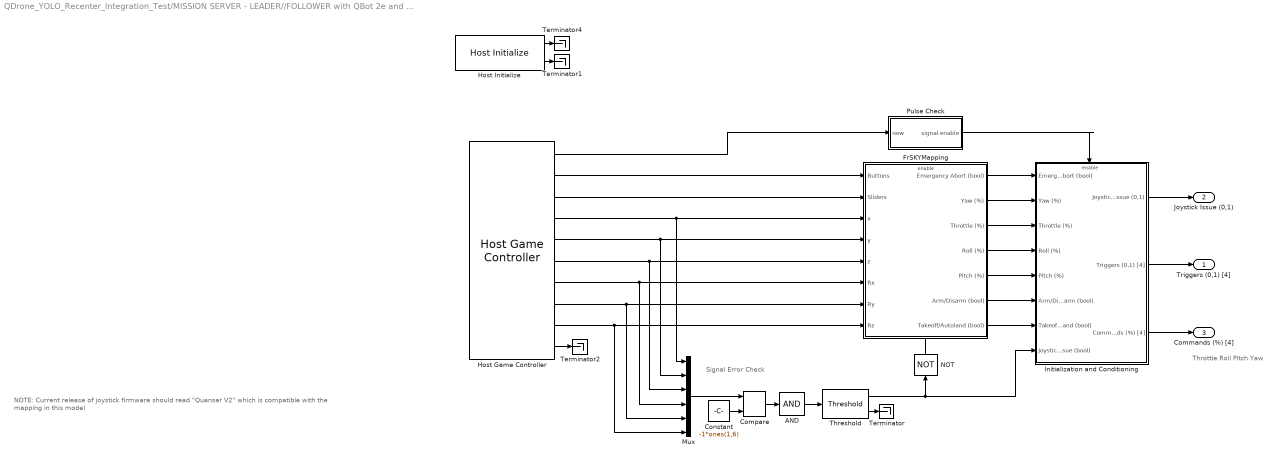
== system QDrone_YOLO_Recenter_Integration_Test/MISSION SERVER - LEADER//FOLLOWER with QBot 2e and QDrone/JOYSTICK ==
  note: Throttle
      | Roll
      | Pitch
      | Yaw
  note: Signal Error Check
  note: NOTE: Current release of joystick firmware should read "Quanser V2" which is compatible with the mapping in this model
  AND : Logic  Inputs=1  AllPortsSameDT=off  OutDataTypeStr=boolean
  Compare : quarc_library/Logic Operations/Compare  operator===  output_data_type=boolean
      settings: SourceProductName=QUARC Targets
  Constant : Constant  Value=-1*ones(1,6)
  FrSKYMapping : Subsystem
  Host Game Controller : quarc_library/Devices/Peripherals/Host/Host Game Controller  object_name=Host-1  controller=1  buffer_size=20  deadzone=[]  saturation=[]  sample_time=qc_get_step_size  auto_center=off  enabled=on  debug_mode=off
      settings: SourceProductName=QUARC Targets
  Host Initialize : quarc_library/Devices/Peripherals/Host/Host Initialize  object_name=Host-1  uri_source=Use external mode communications  uri=tcpip://localhost:18001  send_buffer_size=1000  receive_buffer_size=1000  thread_priority=0  run_client=on  use_window=off  window_position=[]  sample_time=qc_get_step_size  active=on
      settings: SourceProductName=QUARC Targets
  Initialization and Conditioning : Subsystem  TreatAsAtomicUnit=on
  Mux : Mux  Inputs=6
  NOT : Logic  Operator=NOT  IconShape=distinctive  AllPortsSameDT=off  OutDataTypeStr=boolean
  Pulse Check : Subsystem  TreatAsAtomicUnit=on
  Terminator{,1..2,4} (4 alike) : Terminator
  Threshold : quarc_library/Discontinuities/Threshold  operator=>=  param_src=Specify via dialog  threshold=0.5  duration=0.2
      settings: SourceProductName=QUARC Targets
  Triggers (0,1) [4] : Outport  VectorParamsAs1DForOutWhenUnconnected=off
  Joystick Issue (0,1) : Outport  Port=2  VectorParamsAs1DForOutWhenUnconnected=off
  Commands (%) [4] : Outport  Port=3  VectorParamsAs1DForOutWhenUnconnected=off
  wires:
  Initialization and Conditioning/1(Joystick Issue (0,1)) -> Joystick Issue (0,1)/1
  Host Game Controller/10 -> Terminator2/1
  Host Initialize/1 -> Terminator4/1
  Host Initialize/2 -> Terminator1/1
  Initialization and Conditioning/2(Triggers (0,1) [4]) -> Triggers (0,1) [4]/1
  Initialization and Conditioning/3(Commands (%) [4]) -> Commands (%) [4]/1
  AND/1 -> Threshold/1
  NOT/1 -> FrSKYMapping/Enable
  Threshold/1 -> Initialization and Conditioning/8(Joystick Issue (bool)), NOT/1
  Host Game Controller/3 -> FrSKYMapping/2(Sliders)
  Host Game Controller/2 -> FrSKYMapping/1(Buttons)
  Threshold/2 -> Terminator/1
  Compare/1 -> AND/1
  Constant/1 -> Compare/2
  Mux/1 -> Compare/1
  Host Game Controller/9 -> FrSKYMapping/8(Rz), Mux/6
  Host Game Controller/8 -> FrSKYMapping/7(Ry), Mux/5
  Host Game Controller/7 -> FrSKYMapping/6(Rx), Mux/4
  Host Game Controller/6 -> FrSKYMapping/5(z), Mux/3
  Host Game Controller/5 -> FrSKYMapping/4(y), Mux/2
  Host Game Controller/4 -> FrSKYMapping/3(x), Mux/1
  FrSKYMapping/7(Takeoff/Autoland (bool)) -> Initialization and Conditioning/7(Takeoff/AutoLand (bool))
  Pulse Check/1(signal enable) -> Initialization and Conditioning/Enable
  Host Game Controller/1 -> Pulse Check/1(new)
  FrSKYMapping/4(Roll (%)) -> Initialization and Conditioning/4(Roll (%))
  FrSKYMapping/6("Arm/Disarm (bool) ") -> Initialization and Conditioning/6(Arm/Disarm (bool))
  FrSKYMapping/5(Pitch (%)) -> Initialization and Conditioning/5(Pitch (%))
  FrSKYMapping/1(Emergency Abort (bool)) -> Initialization and Conditioning/1(Emergency Abort (bool))
  FrSKYMapping/3(Throttle (%)) -> Initialization and Conditioning/3(Throttle (%))
  FrSKYMapping/2(Yaw (%)) -> Initialization and Conditioning/2(Yaw (%))

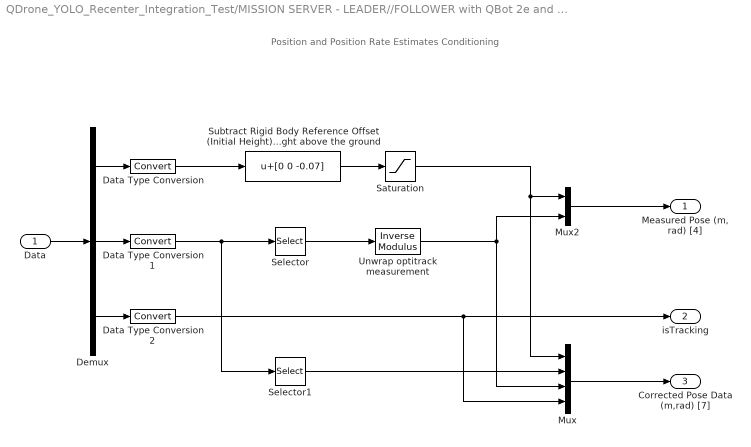
== system QDrone_YOLO_Recenter_Integration_Test/MISSION SERVER - LEADER//FOLLOWER with QBot 2e and QDrone/Measurement Conditioning ==
  note: Position and Position Rate Estimates Conditioning
  Data : Inport
  Data Type Conversion : DataTypeConversion
  Data Type Conversion1 : DataTypeConversion
  Data Type Conversion2 : DataTypeConversion
  Demux : Demux  Outputs=[3 3 1]
  Mux : Mux
  Mux2 : Mux  Inputs=[3 1]
  Saturation : Saturate  UpperLimit=[2 2 5]  LowerLimit=[-2 -2 0]
  Selector : Selector  InputPortWidth=3  IndexOptions=Index vector (dialog)  Indices=[3]  OutputSizes=1
  Selector1 : Selector  InputPortWidth=3  IndexOptions=Index vector (dialog)  Indices=[1 2]  OutputSizes=1
  Subtract Rigid Body Reference Offset (Initial Height) to get height above the ground : Bias  Bias=[0 0 -0.07]
  Unwrap optitrack measurement : quarc_library/Discontinuities/Inverse Modulus  modulus=2*pi  output_derivative=off  output_revolutions=off  max_x=Inf  min_x=-Inf
  "Measured Pose (m, rad) [4]" : Outport  VectorParamsAs1DForOutWhenUnconnected=off
  isTracking : Outport  Port=2  VectorParamsAs1DForOutWhenUnconnected=off
  Corrected Pose Data (m,rad) [7] : Outport  Port=3  VectorParamsAs1DForOutWhenUnconnected=off
  wires:
  Demux/2 -> Data Type Conversion1/1
  Demux/1 -> Data Type Conversion/1
  Demux/3 -> Data Type Conversion2/1
  Mux2/1 -> "Measured Pose (m, rad) [4]"/1
  Data/1 -> Demux/1
  Data Type Conversion2/1 -> Mux/4, isTracking/1
  Subtract Rigid Body Reference Offset (Initial Height) to get height above the ground/1 -> Saturation/1
  Saturation/1 -> Mux2/1, Mux/1
  Data Type Conversion1/1 -> Selector1/1, Selector/1
  Selector/1 -> Unwrap optitrack measurement/1
  Data Type Conversion/1 -> Subtract Rigid Body Reference Offset (Initial Height) to get height above the ground/1
  Unwrap optitrack measurement/1 -> Mux/3, Mux2/2
  Mux/1 -> Corrected Pose Data (m,rad) [7]/1
  Selector1/1 -> Mux/2

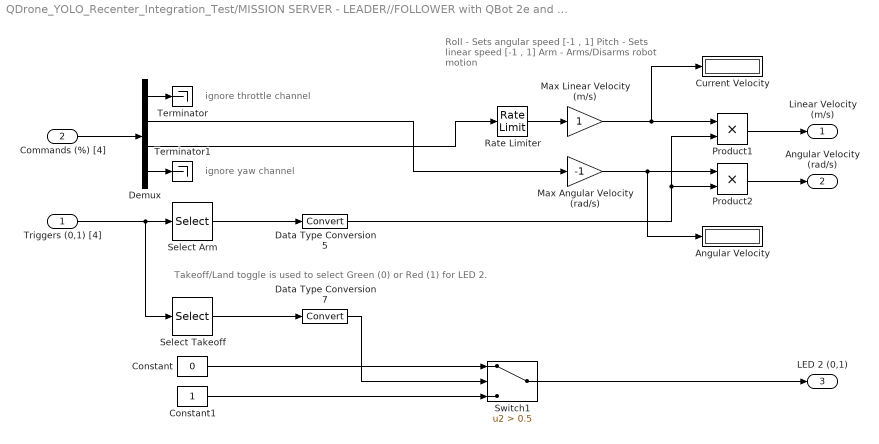
== system QDrone_YOLO_Recenter_Integration_Test/MISSION SERVER - LEADER//FOLLOWER with QBot 2e and QDrone/Raw joystick to Linear and Angular Velocity Commands ==
  note: Takeoff/Land toggle is used to select Green (0) or Red (1) for LED 2.
  note: Roll		- Sets angular speed  	[-1		, 1]
      | Pitch	- Sets linear speed  	[-1		, 1]
      | Arm		- Arms/Disarms robot motion
  note: ignore throttle channel
  note: ignore yaw channel
  Triggers (0,1) [4] : Inport
  Commands (%) [4] : Inport  Port=2
  Angular Velocity : Display
  Constant : Constant  Value=0
  Constant1 : Constant
  Current Velocity : Display
  Data Type Conversion5 : DataTypeConversion
  Data Type Conversion7 : DataTypeConversion
  Demux : Demux
  Max Angular Velocity (rad/s) : Gain  Gain=-1
  Max Linear Velocity (m/s) : Gain
  Product1 : Product
  Product2 : Product
  Rate Limiter : RateLimiter  SampleTimeMode=inherited
  Select Arm : Selector  InputPortWidth=4  IndexOptions=Index vector (dialog)  Indices=[1]  OutputSizes=1
  Select Takeoff : Selector  InputPortWidth=4  IndexOptions=Index vector (dialog)  Indices=[2]  OutputSizes=1
  Switch1 : Switch  Criteria=u2 > Threshold  Threshold=0.5
  Terminator : Terminator
  Terminator1 : Terminator
  Linear Velocity (m/s) : Outport  InitialOutput=0  VectorParamsAs1DForOutWhenUnconnected=off
  Angular Velocity (rad/s) : Outport  Port=2  InitialOutput=0  VectorParamsAs1DForOutWhenUnconnected=off
  LED 2 (0,1) : Outport  Port=3  InitialOutput=0  VectorParamsAs1DForOutWhenUnconnected=off
  wires:
  Commands (%) [4]/1 -> Demux/1
  Select Takeoff/1 -> Data Type Conversion7/1
  Switch1/1 -> LED 2 (0,1)/1
  Triggers (0,1) [4]/1 -> Select Takeoff/1, Select Arm/1
  Data Type Conversion7/1 -> Switch1/2
  Demux/4 -> Terminator1/1
  Data Type Conversion5/1 -> Product1/2, Product2/2
  Demux/3 -> Rate Limiter/1
  Demux/2 -> Max Angular Velocity (rad/s)/1
  Rate Limiter/1 -> Max Linear Velocity (m/s)/1
  Product2/1 -> Angular Velocity (rad/s)/1
  Constant1/1 -> Switch1/3
  Constant/1 -> Switch1/1
  Max Angular Velocity (rad/s)/1 -> Angular Velocity/1, Product2/1
  Product1/1 -> Linear Velocity (m/s)/1
  Demux/1 -> Terminator/1
  Max Linear Velocity (m/s)/1 -> Current Velocity/1, Product1/1
  Select Arm/1 -> Data Type Conversion5/1

== system QDrone_YOLO_Recenter_Integration_Test/MISSION SERVER - LEADER//FOLLOWER with QBot 2e and QDrone/Triggered Subsystem ==
  note: This looks for the first falling edge of the communication issue before allowing a communication issue to be triggered,
      | because the mission server model starts first.
  Trigger : TriggerPort  TriggerType=falling  VariantControl=Variant
  Add : Sum
  Compare To Constant : simulink/Logic and Bit Operations/Compare To Constant  relop=>=  const=1  OutDataTypeStr=boolean
  Constant : Constant
  Memory : Memory  InheritSampleTime=on
  Communication Issue (0,1) : Outport  InitialOutput=0  VectorParamsAs1DForOutWhenUnconnected=off
  wires:
  Constant/1 -> Add/1
  Memory/1 -> Add/2
  Add/1 -> Compare To Constant/1, Memory/1
  Compare To Constant/1 -> Communication Issue (0,1)/1

== system QDrone_YOLO_Recenter_Integration_Test/MISSION SERVER - LEADER//FOLLOWER with QBot 2e and QDrone/Triggered Subsystem1 ==
  note: This looks for the first falling edge of the communication issue before allowing a communication issue to be triggered,
      | because the mission server model starts first.
  Trigger : TriggerPort  TriggerType=falling  VariantControl=Variant
  Add : Sum
  Compare To Constant : simulink/Logic and Bit Operations/Compare To Constant  relop=>=  const=1  OutDataTypeStr=boolean
  Constant : Constant
  Memory : Memory  InheritSampleTime=on
  Communication Issue (0,1) : Outport  InitialOutput=0  VectorParamsAs1DForOutWhenUnconnected=off
  wires:
  Compare To Constant/1 -> Communication Issue (0,1)/1
  Add/1 -> Memory/1, Compare To Constant/1
  Memory/1 -> Add/2
  Constant/1 -> Add/1

== system QDrone_YOLO_Recenter_Integration_Test/MISSION SERVER - LEADER//FOLLOWER with QBot 2e and QDrone/Calculate Home Pose/Enabled Subsystem ==
  "Pose (m, rad ) [4] " : Inport
  Enable : EnablePort
  "Home Pose (m, rad ) [4]" : Outport  VectorParamsAs1DForOutWhenUnconnected=off
  wires:
  "Pose (m, rad ) [4] "/1 -> "Home Pose (m, rad ) [4]"/1

== system QDrone_YOLO_Recenter_Integration_Test/MISSION SERVER - LEADER//FOLLOWER with QBot 2e and QDrone/Data Server (Localization) /Convention Correction (Motive Frame to Research Studio Frame) - QBot 2e ==
  note: MF_R_RSF
  note: This subsystem converts measurements in the Motive Frame (MF)(raw optitrack) into the Research Studio Frame (RSF).
  note: RSF_R_MF
  note: XYZ in MF
  note: RPY in MF
  note: position
  note: attitude
  note: XYZ in RSF
  note: RPY in RSF
  xyz_MF (m) [3] : Inport
  rot_MF (rad) [3] : Inport  Port=2
  Inverse of Orthonormal Matrix is its Transpose : Math  Operator=transpose  SignedPower=on  SaturateOnIntegerOverflow=on
  Prevent Gimbal Lock : Subsystem
  Product : Product  Multiplication=Matrix(*)
  Product1 : Product  Multiplication=Matrix(*)
  Rotate Basis from RSF to MF : Constant  Value=[0 -1 0;0 0 1;-1 0 0]
  xyz_RSF (m) [3] : Outport  VectorParamsAs1DForOutWhenUnconnected=off
  rot_RSF (rad) [3] : Outport  Port=2  VectorParamsAs1DForOutWhenUnconnected=off
  wires:
  Rotate Basis from RSF to MF/1 -> Inverse of Orthonormal Matrix is its Transpose/1
  xyz_MF (m) [3]/1 -> Product1/2
  Inverse of Orthonormal Matrix is its Transpose/1 -> Product1/1, Product/1
  rot_MF (rad) [3]/1 -> Product/2
  Product1/1 -> xyz_RSF (m) [3]/1
  Product/1 -> Prevent Gimbal Lock/1(Attitude (rad) [3])
  Prevent Gimbal Lock/1("Attitude (rad) [3] ") -> rot_RSF (rad) [3]/1

== system QDrone_YOLO_Recenter_Integration_Test/MISSION SERVER - LEADER//FOLLOWER with QBot 2e and QDrone/Data Server (Localization) /Convention Correction (Motive Frame to Research Studio Frame) - QDrone ==
  note: MF_R_RSF
  note: This subsystem converts measurements in the Motive Frame (MF)(raw optitrack) into the Research Studio Frame (RSF).
  note: RSF_R_MF
  note: XYZ in MF
  note: RPY in MF
  note: position
  note: attitude
  note: XYZ in RSF
  note: RPY in RSF
  xyz_MF (m) [3] : Inport
  rot_MF (rad) [3] : Inport  Port=2
  Inverse of Orthonormal Matrix is its Transpose : Math  Operator=transpose  SignedPower=on  SaturateOnIntegerOverflow=on
  Prevent Gimbal Lock : Subsystem
  Product : Product  Multiplication=Matrix(*)
  Product1 : Product  Multiplication=Matrix(*)
  Rotate Basis from RSF to MF : Constant  Value=[0 -1 0;0 0 1;-1 0 0]
  xyz_RSF (m) [3] : Outport  VectorParamsAs1DForOutWhenUnconnected=off
  rot_RSF (rad) [3] : Outport  Port=2  VectorParamsAs1DForOutWhenUnconnected=off
  wires:
  Rotate Basis from RSF to MF/1 -> Inverse of Orthonormal Matrix is its Transpose/1
  xyz_MF (m) [3]/1 -> Product1/2
  Inverse of Orthonormal Matrix is its Transpose/1 -> Product1/1, Product/1
  rot_MF (rad) [3]/1 -> Product/2
  Product1/1 -> xyz_RSF (m) [3]/1
  Product/1 -> Prevent Gimbal Lock/1(Attitude (rad) [3])
  Prevent Gimbal Lock/1("Attitude (rad) [3] ") -> rot_RSF (rad) [3]/1

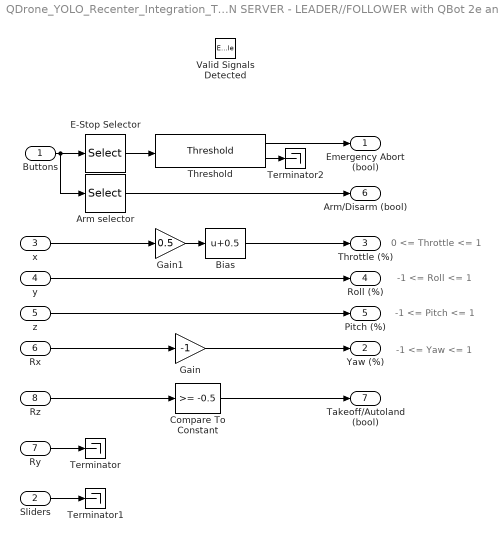
== system QDrone_YOLO_Recenter_Integration_Test/MISSION SERVER - LEADER//FOLLOWER with QBot 2e and QDrone/JOYSTICK/FrSKYMapping ==
  note: -1 <= Pitch <= 1
  note: -1 <= Roll <= 1
  note: 0 <= Throttle <= 1
  note: -1 <= Yaw <= 1
  Buttons : Inport
  Sliders : Inport  Port=2
  x : Inport  Port=3
  y : Inport  Port=4
  z : Inport  Port=5
  Rx : Inport  Port=6
  Ry : Inport  Port=7
  Rz : Inport  Port=8
  Valid Signals Detected : EnablePort
  Arm selector : Selector  InputPortWidth=32  IndexOptions=Index vector (dialog)  Indices=[2]  OutputSizes=1
  Bias : Bias  Bias=0.5
  Compare To Constant : simulink/Logic and Bit Operations/Compare To Constant  relop=>=  const=-0.5  OutDataTypeStr=boolean
  E-Stop Selector : Selector  InputPortWidth=32  IndexOptions=Index vector (dialog)  Indices=[1]  OutputSizes=1
  Gain : Gain  Gain=-1
  Gain1 : Gain  Gain=0.5
  Terminator : Terminator
  Terminator1 : Terminator
  Terminator2 : Terminator
  Threshold : quarc_library/Discontinuities/Threshold  operator=>=  param_src=Specify via dialog  threshold=0.5  duration=0.2
      settings: SourceProductName=QUARC Targets
  Emergency Abort (bool) : Outport  VectorParamsAs1DForOutWhenUnconnected=off
  Yaw (%) : Outport  Port=2  VectorParamsAs1DForOutWhenUnconnected=off
  Throttle (%) : Outport  Port=3  VectorParamsAs1DForOutWhenUnconnected=off
  Roll (%) : Outport  Port=4  VectorParamsAs1DForOutWhenUnconnected=off
  Pitch (%) : Outport  Port=5  VectorParamsAs1DForOutWhenUnconnected=off
  "Arm/Disarm (bool) " : Outport  Port=6  VectorParamsAs1DForOutWhenUnconnected=off
  Takeoff/Autoland (bool) : Outport  Port=7  VectorParamsAs1DForOutWhenUnconnected=off
  wires:
  Bias/1 -> Throttle (%)/1
  Gain1/1 -> Bias/1
  Gain/1 -> Yaw (%)/1
  Threshold/2 -> Terminator2/1
  Threshold/1 -> Emergency Abort (bool)/1
  Compare To Constant/1 -> Takeoff/Autoland (bool)/1
  Rz/1 -> Compare To Constant/1
  E-Stop Selector/1 -> Threshold/1
  Sliders/1 -> Terminator1/1
  Ry/1 -> Terminator/1
  Rx/1 -> Gain/1
  z/1 -> Pitch (%)/1
  y/1 -> Roll (%)/1
  x/1 -> Gain1/1
  Arm selector/1 -> "Arm/Disarm (bool) "/1
  Buttons/1 -> E-Stop Selector/1, Arm selector/1

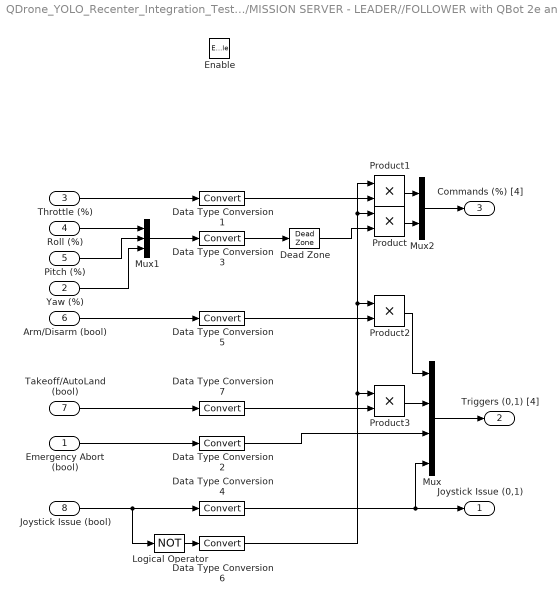
== system QDrone_YOLO_Recenter_Integration_Test/MISSION SERVER - LEADER//FOLLOWER with QBot 2e and QDrone/JOYSTICK/Initialization and Conditioning ==
  Emergency Abort (bool) : Inport
  Yaw (%) : Inport  Port=2
  Throttle (%) : Inport  Port=3
  Roll (%) : Inport  Port=4
  Pitch (%) : Inport  Port=5
  Arm/Disarm (bool) : Inport  Port=6
  Takeoff/AutoLand (bool) : Inport  Port=7
  Joystick Issue (bool) : Inport  Port=8
  Enable : EnablePort  StatesWhenEnabling=reset
  Data Type Conversion{1..7} (7 alike) : DataTypeConversion
  Dead Zone : DeadZone  LowerValue=-0.01  UpperValue=0.01  SaturateOnIntegerOverflow=on
  Logical Operator : Logic  Operator=NOT  AllPortsSameDT=off  OutDataTypeStr=boolean
  Mux : Mux
  Mux1 : Mux  Inputs=3
  Mux2 : Mux  Inputs=2
  Product{,1..3} (4 alike) : Product
  Joystick Issue (0,1) : Outport  InitialOutput=0  VectorParamsAs1DForOutWhenUnconnected=off
  Triggers (0,1) [4] : Outport  Port=2  InitialOutput=0  VectorParamsAs1DForOutWhenUnconnected=off
  Commands (%) [4] : Outport  Port=3  InitialOutput=0  VectorParamsAs1DForOutWhenUnconnected=off
  wires:
  Mux2/1 -> Commands (%) [4]/1
  Data Type Conversion7/1 -> Product3/2
  Product3/1 -> Mux/2
  Takeoff/AutoLand (bool)/1 -> Data Type Conversion7/1
  Data Type Conversion5/1 -> Product2/2
  Product2/1 -> Mux/1
  Data Type Conversion6/1 -> Product3/1, Product2/1, Product/1, Product1/1
  Dead Zone/1 -> Product/2
  Data Type Conversion1/1 -> Product1/2
  Product1/1 -> Mux2/1
  Product/1 -> Mux2/2
  Logical Operator/1 -> Data Type Conversion6/1
  Data Type Conversion2/1 -> Mux/3
  Mux/1 -> Triggers (0,1) [4]/1
  Arm/Disarm (bool)/1 -> Data Type Conversion5/1
  Data Type Conversion3/1 -> Dead Zone/1
  Emergency Abort (bool)/1 -> Data Type Conversion2/1
  Data Type Conversion4/1 -> Joystick Issue (0,1)/1, Mux/4
  Yaw (%)/1 -> Mux1/3
  Pitch (%)/1 -> Mux1/2
  Roll (%)/1 -> Mux1/1
  Throttle (%)/1 -> Data Type Conversion1/1
  Mux1/1 -> Data Type Conversion3/1
  Joystick Issue (bool)/1 -> Logical Operator/1, Data Type Conversion4/1
